simulink model "FCNPC_3_Level_Resonant_Drive_NLM"  (R2023b)
settings: Solver=VariableStepAuto  StartTime=0.0  StopTime=0.002  RelTol=1e-3
libraries: spsMosfetLib x8, spsVoltageMeasurementLib x5, spsSeriesRLCBranchLib x4, spsCurrentMeasurementLib x2, spsMeanLib x2, simulink_extras x2, spsDCVoltageSourceLib x1, spsTHDLib x1, sps_lib x1
settings Model: SimulationMode=accelerator  Creator=abc6820292  LastModifiedBy=Qu
settings DebuggingCC: UnconnectedInputMsg=warning  UnconnectedOutputMsg=warning  UnconnectedLineMsg=warning
settings ModelReferenceCC: EnableRefExpFcnMdlSchedulingChecks=on
settings RTWCC: DLArmComputeVersion=19.05

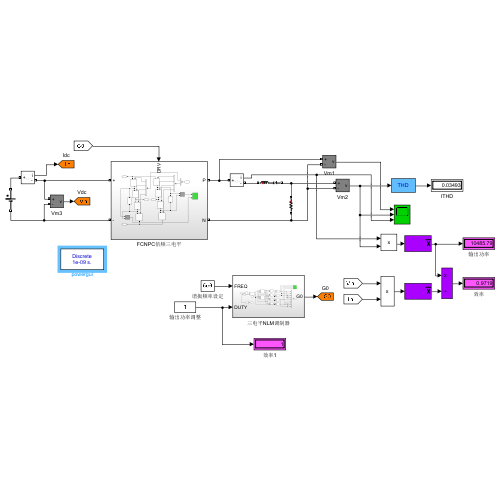
[thumbnail: Simulink's stored preview of the top-level diagram]
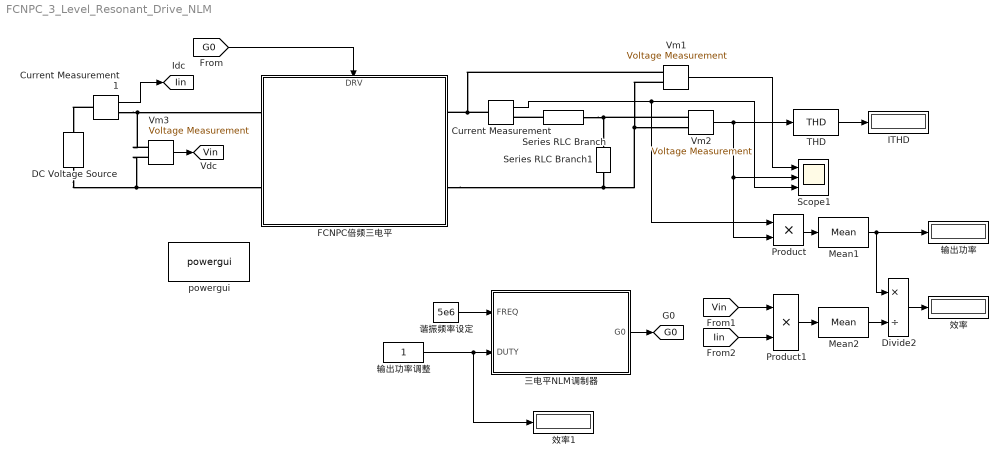
== system FCNPC_3_Level_Resonant_Drive_NLM ==
  Current Measurement : spsCurrentMeasurementLib/Current Measurement  PhasorSimulation=off  OutputType=Complex  PSBequivalent=0
  Current Measurement1 : spsCurrentMeasurementLib/Current Measurement  PhasorSimulation=off  OutputType=Complex  PSBequivalent=0
  DC Voltage Source : spsDCVoltageSourceLib/DC Voltage Source  Amplitude=700  Measurements=None
  Divide2 : Product  Inputs=*/
  FCNPC倍频三电平 : Subsystem
      settings: PortSchema="{\"entries\":[{\"content\":{\"sides\":[{\"content\":{\"connectorIds\":[\"LConn1\",\"LConn2\"]},\"type\":\"ConnectorPlacement.EquallySpacedRectSide\",\"uuid\":\"398c122b-42ab-47b5-90f5-37fce70dd24f\"},{\"content\":{\"connectorIds\":[\"RConn1\",\"RConn2\"],\"side\":\"RIGHT\"},\"type\":\"ConnectorPlacement.EquallySpacedRectSide\",\"uuid\":\"ed207fa5-4e2f-4512-9e54-1ade019b37db\"},{\"content\":{\"connectorIds\":[\"In1\"],\"side\":\"TOP\"},\"type\":\"ConnectorPlacement.EquallySpacedRectSide\",\"uuid\":\"4f98c6d3-8f23-4a23-9b67-30b66988ab08\"}]},\"type\":\"ConnectorPlacement.EquallySpacedConnector\",\"uuid\":\"adb2c5a8-768b-4e9c-a829-cef28d4f8aed\"}],\"packageUris\":[\"http://schema.mathworks.com/mf0/Connector/R2020b\"],\"version\":\"1.0\"}"
  ITHD : Display
  Mean1 : spsMeanLib/Mean  Freq=5e5  Vinit=0  Ts=0
  Mean2 : spsMeanLib/Mean  Freq=5e5  Vinit=0  Ts=0
  Product : Product
  Product1 : Product
  Scope1 : Scope  NumInputPorts=3
  Series RLC Branch : spsSeriesRLCBranchLib/Series RLC Branch  LConnTagsString=__new0  RConnTagsString=__new0  BranchType=LC  Resistance=1  Inductance=1e-6  SetiL0=off  InitialCurrent=0  Capacitance=1e-9  Setx0=off  InitialVoltage=0  Measurements=None
  Series RLC Branch1 : spsSeriesRLCBranchLib/Series RLC Branch  LConnTagsString=__new0  RConnTagsString=__new0  BranchType=R  Resistance=9  Inductance=0.1  SetiL0=off  InitialCurrent=0  Capacitance=1e-4  Setx0=off  InitialVoltage=0  Measurements=None
  THD : spsTHDLib/THD  Freq=5e6  Ts=0
  Vm1 : spsVoltageMeasurementLib/Voltage Measurement  PhasorSimulation=off  OutputType=Complex  PSBequivalent=0
  Vm2 : spsVoltageMeasurementLib/Voltage Measurement  PhasorSimulation=off  OutputType=Complex  PSBequivalent=0
  Vm3 : spsVoltageMeasurementLib/Voltage Measurement  PhasorSimulation=off  OutputType=Complex  PSBequivalent=0
  powergui : sps_lib/powergui  Priority=1  SimulationMode=Discrete  SampleTime=1e-9  frequency=60  Iterations=50  frequencyindice=0  Pbase=100e6  ErrMax=1e-4  UnitsV=kV  UnitsW=MW  buscounter=0  FunctionMessages=off  echomessages=off  EnableUseOfTLC=off  CurrentSourceSwitches=off  DisableSnubberDevices=off  DisableRonSwitches=off  DisableVfSwitches=off  DisplayEquations=off  AutomaticDiscreteSolvers=off  SolverType=Tustin/Backward Euler (TBE)  Interpol=off  ExternalGateDelay=off  methode=off  Ts=100  x0status=blocks  SPID=on  SwTol=0  HookPort=off  NonlinearTolerance=1e-4  nMaxIteration=100  ContinueOnMaxIteration=off  RestoreLinks=warning  ResistiveCurrentMeasurement=off  Frange=[0:2:500]  Ylog=off  Xlog=on  ShowGrid=off  save=off  variable=ZData  structure=0  ZoomFFT=off  StartTime=0.0  cycles=1  DisplayStyle=1  fundamental=60  FreqAxis=off  MaxFrequency=1000  frequencyindicesteady=1  RmsSteady=1  display=off
  三电平NLM调制器 : Subsystem
  效率 : Display
  效率1 : Display
  谐振频率设定 : Constant  Value=5e6
  输出功率 : Display
      settings: Format=bank
  输出功率调整 : Constant
  tag scope: G0=global, Iin=global, Vin=global
  wires:
  Vm1/1 -> Scope1/1
  三电平NLM调制器/1(G0) -> [G0]
  [G0] -> FCNPC倍频三电平/1(DRV)
  谐振频率设定/1 -> 三电平NLM调制器/1(FREQ)
  Vm2/1 -> Scope1/2, Product/2, THD/1
  THD/1 -> ITHD/1
  Current Measurement/1 -> Product/1, Scope1/3
  Current Measurement1/1 -> [Iin]
  Vm3/1 -> [Vin]
  输出功率调整/1 -> 三电平NLM调制器/2(DUTY), 效率1/1
  Product/1 -> Mean1/1
  Product1/1 -> Mean2/1
  Mean1/1 -> Divide2/1, 输出功率/1
  Mean2/1 -> Divide2/2
  Divide2/1 -> 效率/1
  [Vin] -> Product1/1
  [Iin] -> Product1/2
  connections:
  Series RLC Branch/LConn1 -- Current Measurement/RConn1
  Series RLC Branch1/RConn1 -- FCNPC倍频三电平/RConn2 -- Vm1/LConn2 -- Vm2/LConn2
  Series RLC Branch/RConn1 -- Series RLC Branch1/LConn1 -- Vm2/LConn1
  Current Measurement1/RConn1 -- Vm3/LConn1 -- FCNPC倍频三电平/LConn1
  Current Measurement1/LConn1 -- DC Voltage Source/RConn1
  DC Voltage Source/LConn1 -- Vm3/LConn2 -- FCNPC倍频三电平/LConn2
  Vm1/LConn1 -- FCNPC倍频三电平/RConn1 -- Current Measurement/LConn1

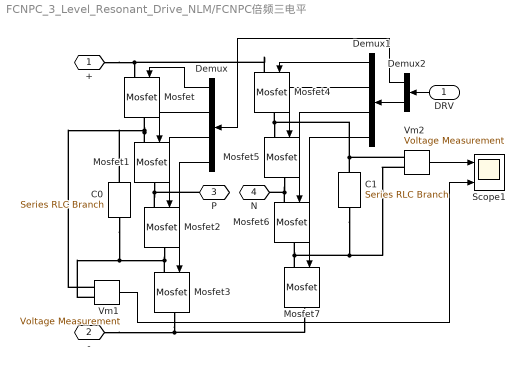
== system FCNPC_3_Level_Resonant_Drive_NLM/FCNPC倍频三电平 ==
  DRV : Inport
  C0 : spsSeriesRLCBranchLib/Series RLC Branch  LConnTagsString=__new0  RConnTagsString=__new0  BranchType=C  Resistance=0.05  Inductance=6e-4  SetiL0=off  InitialCurrent=0  Capacitance=1e-3  Setx0=on  InitialVoltage=350  Measurements=None
  C1 : spsSeriesRLCBranchLib/Series RLC Branch  LConnTagsString=__new0  RConnTagsString=__new0  BranchType=C  Resistance=0.05  Inductance=6e-4  SetiL0=off  InitialCurrent=0  Capacitance=1e-3  Setx0=on  InitialVoltage=350  Measurements=None
  Demux : Demux
  Demux1 : Demux
  Demux2 : Demux  Outputs=2
  Mosfet{,1..7} (8 alike) : spsMosfetLib/Mosfet  Ron=0.03  Lon=0  Rd=0.01  Vfd=0  IC=0  Rs=1000  Cs=1e-9  Measurements=off
  Scope1 : Scope  NumInputPorts=2
  Vm1 : spsVoltageMeasurementLib/Voltage Measurement  PhasorSimulation=off  OutputType=Complex  PSBequivalent=0
  Vm2 : spsVoltageMeasurementLib/Voltage Measurement  PhasorSimulation=off  OutputType=Complex  PSBequivalent=0
  + : PMIOPort  Side=Left
  - : PMIOPort  Port=2  Side=Left
  P : PMIOPort  Port=3  Side=Right
  N : PMIOPort  Port=4  Side=Right
  wires:
  Demux/3 -> Mosfet2/1
  Demux2/1 -> Demux/1
  Demux1/4 -> Mosfet7/1
  Demux1/2 -> Mosfet5/1
  Demux/4 -> Mosfet3/1
  Demux/1 -> Mosfet/1
  Demux1/3 -> Mosfet6/1
  Demux1/1 -> Mosfet4/1
  Demux2/2 -> Demux1/1
  DRV/1 -> Demux2/1
  Demux/2 -> Mosfet1/1
  Vm2/1 -> Scope1/1
  Vm1/1 -> Scope1/2
  connections:
  C1/LConn1 -- Vm2/LConn1 -- Mosfet4/RConn1 -- Mosfet5/LConn1
  C0/RConn1 -- Vm1/LConn2 -- Mosfet3/LConn1 -- Mosfet2/RConn1
  P/RConn1 -- Mosfet1/RConn1 -- Mosfet2/LConn1
  Mosfet/RConn1 -- Mosfet1/LConn1 -- C0/LConn1 -- Vm1/LConn1
  C1/RConn1 -- Mosfet7/LConn1 -- Mosfet6/RConn1 -- Vm2/LConn2
  Mosfet5/RConn1 -- Mosfet6/LConn1 -- N/RConn1
  Mosfet/LConn1 -- Mosfet4/LConn1 -- +/RConn1
  -/RConn1 -- Mosfet7/RConn1 -- Mosfet3/RConn1

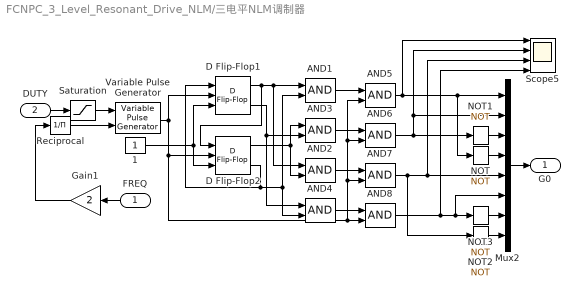
== system FCNPC_3_Level_Resonant_Drive_NLM/三电平NLM调制器 ==
  FREQ : Inport
  DUTY : Inport  Port=2
  1 : Constant
  AND{1..8} (8 alike) : Logic  IconShape=distinctive  AllPortsSameDT=off  OutDataTypeStr=boolean
  D Flip-Flop1 : simulink_extras/Flip Flops/D Flip-Flop
  D Flip-Flop2 : simulink_extras/Flip Flops/D Flip-Flop
  Gain1 : Gain  Gain=2
  Mux2 : Mux  Inputs=8
  NOT{,1..3} (4 alike) : Logic  Operator=NOT  IconShape=distinctive  AllPortsSameDT=off  OutDataTypeStr=boolean
  Reciprocal : Product  Inputs=/
  Saturation : Saturate  UpperLimit=0.9  LowerLimit=0
  Scope5 : Scope  NumInputPorts=4
  Variable Pulse Generator : VariablePulseGenerator  SampleTime=0.1
  G0 : Outport
  wires:
  Reciprocal/1 -> Variable Pulse Generator/2
  1/1 -> D Flip-Flop2/3, D Flip-Flop1/3
  D Flip-Flop1/1 -> D Flip-Flop2/1, AND2/1, AND1/1
  Variable Pulse Generator/1 -> D Flip-Flop1/2, AND5/2, AND6/2, AND7/2, AND8/2, D Flip-Flop2/2
  Mux2/1 -> G0/1
  D Flip-Flop2/1 -> AND3/1, AND2/2
  D Flip-Flop2/2 -> AND1/2, AND4/2, D Flip-Flop1/1
  D Flip-Flop1/2 -> AND4/1, AND3/2
  AND1/1 -> AND5/1
  AND4/1 -> AND8/1
  AND5/1 -> NOT/1, Mux2/1, Scope5/1
  AND6/1 -> NOT1/1, Mux2/2, Scope5/2
  AND7/1 -> Mux2/5, Scope5/3, NOT2/1
  AND8/1 -> Mux2/6, NOT3/1, Scope5/4
  NOT/1 -> Mux2/4
  NOT1/1 -> Mux2/3
  NOT2/1 -> Mux2/8
  NOT3/1 -> Mux2/7
  AND3/1 -> AND6/1
  AND2/1 -> AND7/1
  FREQ/1 -> Gain1/1
  Gain1/1 -> Reciprocal/1
  DUTY/1 -> Saturation/1
  Saturation/1 -> Variable Pulse Generator/1
